simulink model "pendulum_PID"  (R2026a)
settings: Solver=VariableStepAuto  StopTime=15
values from neighbouring files (symbols this model uses):
  Kd_pos = 0    [init_pendulum.m]
  Kd_theta = 0.2    [init_pendulum.m]
  Ki_vel = 0.3    [init_pendulum.m]
  Kp_pos = 0.05    [init_pendulum.m]
  Kp_theta = 2    [init_pendulum.m]
  Kp_vel = 0.25    [init_pendulum.m]
  Kp_yaw = 0.02    [init_pendulum.m]
  manualMode = 0    [init_pendulum.m]
  p = [ ... (first row only)    [init_pendulum.m]
  posRef = 0    [init_pendulum.m]
  q0 = [ ... (first row only)    [init_pendulum.m]
  qd0 = [ ... (first row only)    [init_pendulum.m]
  tauDiffMax = 0.2    [init_pendulum.m]
  tauMax = 2    [init_pendulum.m]
  thetaMax = deg2rad(8)    [init_pendulum.m]
  vMax = 0.2    [init_pendulum.m]
settings Model: Creator=vb  LastModifiedBy=vb

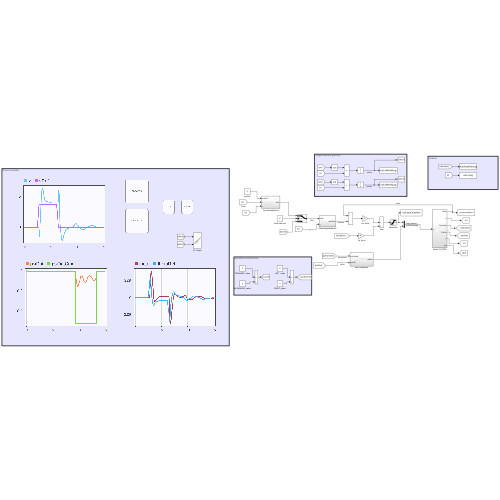
[thumbnail: Simulink's stored preview of the top-level diagram]
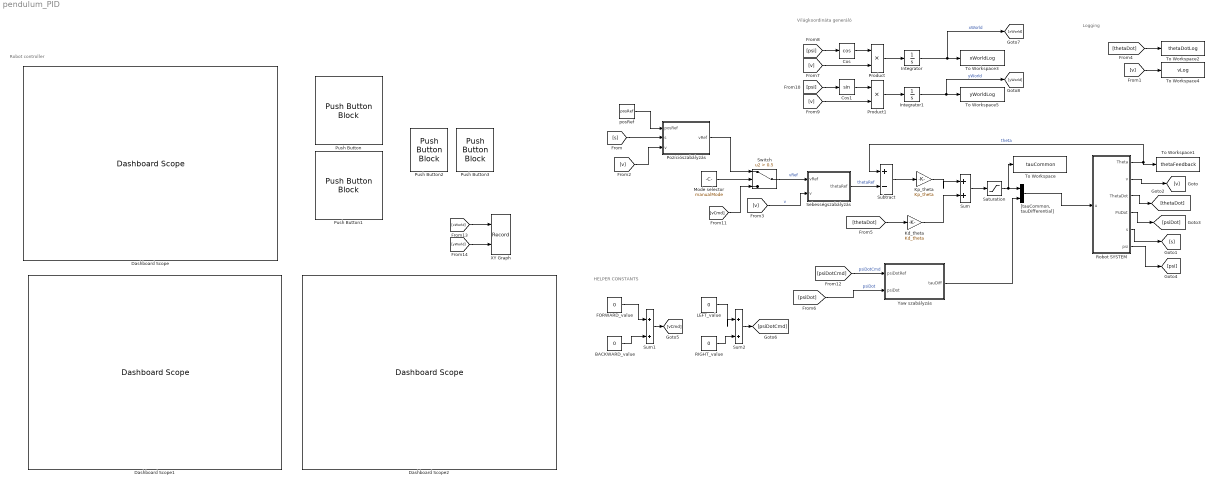
== system pendulum_PID ==
  note: HELPER CONSTANTS
  note: Robot controller
  note: Világkoordináta generáló
  note: Logging
  BACKWARD_value : Constant  Value=0
  Cos : Trigonometry  Operator=cos
  Cos1 : Trigonometry
  Dashboard Scope : DashboardScope  FontColor=[0.0, 0.0, 0.0]
  Dashboard Scope1 : DashboardScope  FontColor=[0.0, 0.0, 0.0]
  Dashboard Scope2 : DashboardScope  FontColor=[0.0, 0.0, 0.0]
  FORWARD_value : Constant  Value=0
  Integrator : Integrator
  Integrator1 : Integrator
  Kd_theta : Gain  Gain=Kd_theta
  Kp_theta : Gain  Gain=Kp_theta
  LEFT_value : Constant  Value=0
  Mode selector : Constant  Value=manualMode
  Pozíciószabályzás : Subsystem
  Product : Product
  Product1 : Product
  Push Button : PushButtonBlock  ButtonText=FORWARD  OnValue=0.15  IconOnColor=[0.0, 0.39215686274509803, 0.0]  IconOffColor=[0.0, 1.0, 0.0]  OffValue=0.000000
  Push Button1 : PushButtonBlock  ButtonText=BACKWARD  OnValue=-0.15  IconOnColor=[0.0, 0.39215686274509803, 0.0]  IconOffColor=[0.0, 1.0, 0.0]  OffValue=0.000000
  Push Button2 : PushButtonBlock  ButtonText=LEFT  OnValue=+0.5236  IconOnColor=[0.0, 0.39215686274509803, 0.0]  IconOffColor=[0.0, 1.0, 0.0]  OffValue=0.000000
  Push Button3 : PushButtonBlock  ButtonText=RIGHT  OnValue=-0.5236  IconOnColor=[0.0, 0.39215686274509803, 0.0]  IconOffColor=[0.0, 1.0, 0.0]  OffValue=0.000000
  RIGHT_value : Constant  Value=0
  Robot SYSTEM : Subsystem
  Saturation : Saturate  UpperLimit=tauMax  LowerLimit=-tauMax
  Sebességszabályzás : Subsystem
  Subtract : Sum  Inputs=+-
  Sum : Sum  Inputs=|++
  Sum1 : Sum  Inputs=|++
  Sum2 : Sum  Inputs=|++
  Switch : Switch  Criteria=u2 > Threshold  Threshold=0.5  SaturateOnIntegerOverflow=off  InputSameDT=off
  To Workspace : ToWorkspace  VariableName=tauCommon  SaveFormat=Timeseries  SampleTime=-1
  To Workspace1 : ToWorkspace  VariableName=thetaFeedback  SaveFormat=Timeseries  SampleTime=-1
  To Workspace2 : ToWorkspace  VariableName=thetaDotLog  SaveFormat=Timeseries  SampleTime=-1
  To Workspace3 : ToWorkspace  VariableName=xWorldLog  SaveFormat=Timeseries  SampleTime=-1
  To Workspace4 : ToWorkspace  VariableName=vLog  SaveFormat=Timeseries  SampleTime=-1
  To Workspace5 : ToWorkspace  VariableName=yWorldLog  SaveFormat=Timeseries  SampleTime=-1
  XY Graph : Record  NumPorts=2.0  FileSettingsInternal="{\"entries\":[{\"content\":{\"excelSettings\":{\"content\":{},\"type\":\"Streamout.ExcelSettings\"},\"parquetSettings\":{\"content\":{},\"type\":\"Streamout.ParquetSettings\"}},\"type\":\"Streamout.FileSettingStorage\",\"uuid\":\"\"}],\"packageUris\":[\"http:\\/\\/schema.mathworks.com\\/mf0\\/streamout_blocks\\/R2020a\"],\"version\":\"1.0\"}"  FrameSettings=[0, 0]  Layout=[1 1]  SignalsInternal="{\"entries\":[{\"content\":{\"signals\":[{\"content\":{\"blockPath\":[],\"dimensions\":[1],\"domain\":\"\",\"lineColor\":\"#a2142f\",\"plots\":[ 1 ],\"port\":1,\"sid\":[\"\"],\"signalID\":1,\"signalName\":\"From13\"},\"type\":\"RecordBlkView.Signal\",\"uuid\":\"\"},{\"content\":{\"blockPath\":[],\"dimensions\":[1],\"domain\":\"\",\"lineColor\":\"#139fff\",\"plots\":[ 1 ],\"port\":2,\"sid\":[\"\"],\"signalID\":2,\"signalName\":\"From14\"},\"type\":\"RecordBlkView.Signal\",\"uuid\":\"\"}]},\"type\":\"RecordBlkView.InputSignals\",\"uuid\":\"\"}],\"packageUris\":[\"http:\\/\\/schema.mathworks.com\\/mf0\\/streamout_blocks\\/R2020a\"],\"version\":\"1.0\"}"  VisualizationBindings="{\"xyplotplugin\":{\"info\":[{\"series\":[{\"bindingParametersList\":[{\"parameter\":\"X-Axis\",\"signalID\":1,\"signalName\":\"From13\"},{\"parameter\":\"Y-Axis\",\"signalID\":2,\"signalName\":\"From14\"}],\"seriesID\":0}],\"subplotID\":1}]}}"  CompatibilityTag=XY
  Yaw szabályzás : Subsystem
  "[tauCommon, tauDifferential]" : Mux  Inputs=2
  posRef : Constant  Value=posRef
  wires:
  Robot SYSTEM/1(Theta) -> To Workspace1/1, Subtract/1  "theta"
  Subtract/1 -> Kp_theta/1
  Kp_theta/1 -> Sum/1
  Kd_theta/1 -> Sum/2
  "[tauCommon, tauDifferential]"/1 -> Robot SYSTEM/1(u)
  Sum/1 -> Saturation/1
  Saturation/1 -> To Workspace/1, "[tauCommon, tauDifferential]"/1
  Robot SYSTEM/2(v) -> [v]
  [v] -> To Workspace4/1
  Robot SYSTEM/5(s) -> [s]
  Sebességszabályzás/1(thetaRef) -> Subtract/2  "thetaRef"
  [v] -> Sebességszabályzás/2(v)  "v"
  [s] -> Pozíciószabályzás/2(s)
  posRef/1 -> Pozíciószabályzás/1(posRef)
  [v] -> Pozíciószabályzás/3(v)
  Robot SYSTEM/3(ThetaDot) -> [thetaDot]
  [thetaDot] -> To Workspace2/1
  [thetaDot] -> Kd_theta/1
  Robot SYSTEM/4(PsiDot) -> [psiDot]
  [psiDot] -> Yaw szabályzás/2(psiDot)  "psiDot"
  Yaw szabályzás/1(tauDiff) -> "[tauCommon, tauDifferential]"/2
  Robot SYSTEM/6(psi) -> [psi]
  Cos/1 -> Product/1
  [v] -> Product/2
  [psi] -> Cos/1
  Product/1 -> Integrator/1
  Integrator/1 -> [xWorld], To Workspace3/1  "xWorld"
  Integrator1/1 -> [yWorld], To Workspace5/1  "yWorld"
  Cos1/1 -> Product1/1
  [psi] -> Cos1/1
  Product1/1 -> Integrator1/1
  [v] -> Product1/2
  Pozíciószabályzás/1(vRef) -> Switch/1
  [vCmd] -> Switch/3
  Switch/1 -> Sebességszabályzás/1(vRef)  "vRef"
  Mode selector/1 -> Switch/2
  FORWARD_value/1 -> Sum1/1
  BACKWARD_value/1 -> Sum1/2
  Sum1/1 -> [vCmd]
  Sum2/1 -> [psiDotCmd]
  LEFT_value/1 -> Sum2/1
  RIGHT_value/1 -> Sum2/2
  [psiDotCmd] -> Yaw szabályzás/1(psiDotRef)  "psiDotCmd"
  [xWorld] -> XY Graph/1
  [yWorld] -> XY Graph/2

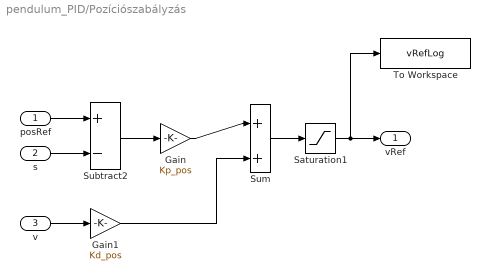
== system pendulum_PID/Pozíciószabályzás ==
  posRef : Inport
  s : Inport  Port=2
  v : Inport  Port=3
  Gain : Gain  Gain=Kp_pos
  Gain1 : Gain  Gain=Kd_pos
  Saturation1 : Saturate  UpperLimit=vMax  LowerLimit=-vMax
  Subtract2 : Sum  Inputs=+-
  Sum : Sum  Inputs=|++
  To Workspace : ToWorkspace  VariableName=vRefLog  SaveFormat=Timeseries  SampleTime=-1
  vRef : Outport
  wires:
  Subtract2/1 -> Gain/1
  Saturation1/1 -> To Workspace/1, vRef/1
  s/1 -> Subtract2/2
  posRef/1 -> Subtract2/1
  v/1 -> Gain1/1
  Sum/1 -> Saturation1/1
  Gain/1 -> Sum/1
  Gain1/1 -> Sum/2

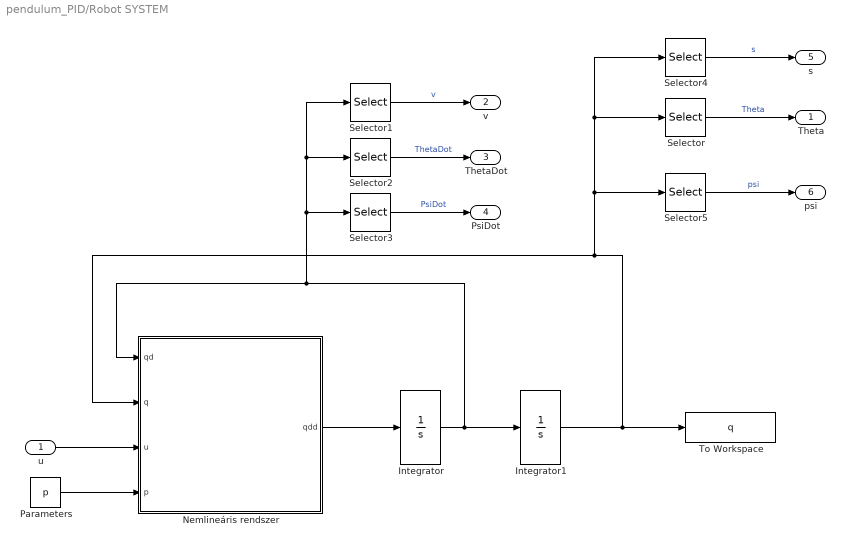
== system pendulum_PID/Robot SYSTEM ==
  u : Inport
  Integrator : Integrator  InitialCondition=qd0
  Integrator1 : Integrator  InitialCondition=q0
  Nemlineáris rendszer : MATLAB Function  TreatAsAtomicUnit=on
  Parameters : Constant  Value=p
  Selector : Selector  InputPortWidth=3  IndexOptions=Index vector (dialog)  Indices=2  OutputSizes=1
  Selector1 : Selector  InputPortWidth=3  IndexOptions=Index vector (dialog)  Indices=1  OutputSizes=1
  Selector2 : Selector  InputPortWidth=3  IndexOptions=Index vector (dialog)  Indices=2  OutputSizes=1
  Selector3 : Selector  InputPortWidth=3  IndexOptions=Index vector (dialog)  Indices=3  OutputSizes=1
  Selector4 : Selector  InputPortWidth=3  IndexOptions=Index vector (dialog)  Indices=1  OutputSizes=1
  Selector5 : Selector  InputPortWidth=3  IndexOptions=Index vector (dialog)  Indices=3  OutputSizes=1
  To Workspace : ToWorkspace  VariableName=q  SaveFormat=Timeseries  SampleTime=-1
  Theta : Outport
  v : Outport  Port=2
  ThetaDot : Outport  Port=3
  PsiDot : Outport  Port=4
  s : Outport  Port=5
  psi : Outport  Port=6
  wires:
  Selector/1 -> Theta/1  "Theta"
  Integrator1/1 -> To Workspace/1, Selector5/1, Selector/1, Selector4/1, Nemlineáris rendszer/2(q)
  Selector1/1 -> v/1  "v"
  Nemlineáris rendszer/1(qdd) -> Integrator/1
  u/1 -> Nemlineáris rendszer/3(u)
  Selector2/1 -> ThetaDot/1  "ThetaDot"
  Selector3/1 -> PsiDot/1  "PsiDot"
  Parameters/1 -> Nemlineáris rendszer/4(p)
  Integrator/1 -> Selector2/1, Selector1/1, Selector3/1, Nemlineáris rendszer/1(qd), Integrator1/1
  Selector4/1 -> s/1  "s"
  Selector5/1 -> psi/1  "psi"

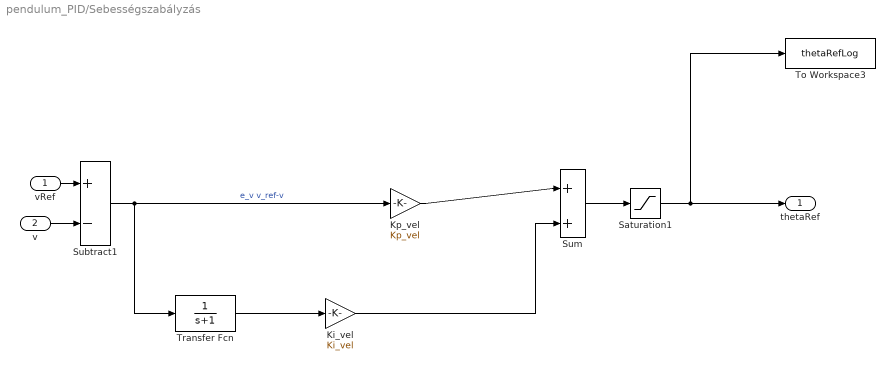
== system pendulum_PID/Sebességszabályzás ==
  vRef : Inport
  v : Inport  Port=2
  Ki_vel : Gain  Gain=Ki_vel
  Kp_vel : Gain  Gain=Kp_vel
  Saturation1 : Saturate  UpperLimit=thetaMax  LowerLimit=-thetaMax
  Subtract1 : Sum  Inputs=+-
  Sum : Sum  Inputs=|++
  To Workspace3 : ToWorkspace  VariableName=thetaRefLog  SaveFormat=Timeseries  SampleTime=-1
  Transfer Fcn : TransferFcn  Denominator=[1 1]
  thetaRef : Outport
  wires:
  v/1 -> Subtract1/2
  Saturation1/1 -> thetaRef/1, To Workspace3/1
  Subtract1/1 -> Transfer Fcn/1, Kp_vel/1  "e_v v_ref-v"
  vRef/1 -> Subtract1/1
  Sum/1 -> Saturation1/1
  Kp_vel/1 -> Sum/1
  Ki_vel/1 -> Sum/2
  Transfer Fcn/1 -> Ki_vel/1

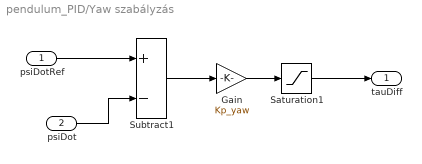
== system pendulum_PID/Yaw szabályzás ==
  psiDotRef : Inport
  psiDot : Inport  Port=2
  Gain : Gain  Gain=Kp_yaw
  Saturation1 : Saturate  UpperLimit=tauDiffMax  LowerLimit=-tauDiffMax
  Subtract1 : Sum  Inputs=+-
  tauDiff : Outport
  wires:
  Gain/1 -> Saturation1/1
  psiDot/1 -> Subtract1/2
  Subtract1/1 -> Gain/1
  Saturation1/1 -> tauDiff/1
  psiDotRef/1 -> Subtract1/1

== matlab function pendulum_PID/Robot SYSTEM/Nemlineáris rendszer ==
  data: qd input; q input; u input; qdd output; p input
function qdd = nonlinearDynamics(qd, q, u, p)

% q  = [s, theta, psi]
% qd = [v, thetaDot, psiDot]
% u  = [tauCommon, tauDifferential]

%% Alap fizikai paraméterek

mb  = p(1);
mw  = p(2);
r   = p(3);
b   = p(4);
l   = p(5);

Ix  = p(6);
Iy  = p(7);
Iz  = p(8);

Ja  = p(9);
Jzw = p(10);

g   = p(11);

%% Súrlódási / veszteségi paraméterek

cMotor   = p(12);   % motor+csapágy viszkózus súrlódás [Nms/rad]
tauMotor = p(13);   % motor+csapágy Coulomb súrlódás [Nm]

cRoll    = p(14);   % gördülési viszkózus ellenállás [Ns/m]
FRoll    = p(15);   % gördülési Coulomb jellegű ellenállás [N]

cAir     = p(16);   % légellenállási együttható

vEps     = p(17);   % simítási sebesség [m/s]
omegaEps = p(18);   % simítási szögsebesség [rad/s]


%% Állapotok

v        = qd(1);
theta    = q(2);
thetaDot = qd(2);
psiDot   = qd(3);


%% Összevont tehetetlenségek

A = mb + 2*mw + 2*Ja/r^2;

C = Iy + mb*l^2;

D = Ix*sin(theta)^2 ...
  + Iz*cos(theta)^2 ...
  + mb*l^2*sin(theta)^2 ...
  + mw*b^2/2 ...
  + Ja*b^2/(2*r^2) ...
  + 2*Jzw;

Dp = 2*sin(theta)*cos(theta) ...
   * (Ix - Iz + mb*l^2);


%% Tömegmátrix

M = [
    A,                  mb*l*cos(theta), 0;
    mb*l*cos(theta),    C,               0;
    0,                  0,               D
];


%% Nemlineáris konzervatív tagok

h = [
    -mb*l*sin(theta)*thetaDot^2;
    -0.5*Dp*psiDot^2 - mb*g*l*sin(theta);
    Dp*thetaDot*psiDot
];


%% Bemeneti mátrix

B = [
     2/r, 0;
    -2,   0;
     0,   b/r
];


%% ------------------------------------------------------------
% Keréksebességek
% ------------------------------------------------------------

vL = v - b/2*psiDot;
vR = v + b/2*psiDot;

omegaL = vL/r;
omegaR = vR/r;


%% ------------------------------------------------------------
% Motor / csapágy relatív szögsebességek
% ------------------------------------------------------------

alphaDotL = omegaL - thetaDot;
alphaDotR = omegaR - thetaDot;


%% ------------------------------------------------------------
% Motor + csapágy súrlódási nyomaték
% ------------------------------------------------------------

tauFricL = cMotor*alphaDotL ...
         + tauMotor*tanh(alphaDotL/omegaEps);

tauFricR = cMotor*alphaDotR ...
         + tauMotor*tanh(alphaDotR/omegaEps);


% közös / különbségi komponensek

tauFricCommon = (tauFricL + tauFricR)/2;
tauFricDiff   = (tauFricR - tauFricL)/2;

uFric = [
    tauFricCommon;
    tauFricDiff
];

QmotorFric = -B*uFric;


%% ------------------------------------------------------------
% Gördülési ellenállás
% ------------------------------------------------------------

FrollL = cRoll*vL ...
       + FRoll*tanh(vL/vEps);

FrollR = cRoll*vR ...
       + FRoll*tanh(vR/vEps);

Qroll = [
    -(FrollL + FrollR);
     0;
    -b/2*(FrollR - FrollL)
];


%% ------------------------------------------------------------
% Légellenállás
% ------------------------------------------------------------

Fair = cAir*v*abs(v);

Qair = [
    -Fair;
     0;
     0
];


%% ------------------------------------------------------------
% Teljes disszipatív általánosított erő
% ------------------------------------------------------------

Qfriction = QmotorFric + Qroll + Qair;


%% ------------------------------------------------------------
% Mozgásegyenlet
% ------------------------------------------------------------

qdd = M \ (B*u + Qfriction - h);

end
